simulink model "Guidance_HIL_XPlane"  (R2026b)
settings: Solver=ode4  StopTime=80  FixedStep=0.005  MaxStep=0.05  MinStep=1e-8  AbsTol=1e-4
StartFcn:
  | ins_initial_state_xplane;
undefined symbols (not defined in the file or in its folder): sensors
(part 2 of 2)

== matlab function Guidance_HIL_XPlane/Navigation/Error_Modeling/GPSNEO8M1/MATLAB Function ==
  data: pos_ned_true input; pos_em output; vel_ned_true input; t input; noise_pos_m input; noise_vel_ms input; w_bias_pos input; vel_em output
function [pos_em, vel_em] = gps_core(pos_ned_true, vel_ned_true, t, ...
    noise_pos_m, noise_vel_ms, w_bias_pos)
%#codegen

coder.extrinsic('ins_gps_measurements');
coder.extrinsic('evalin');

sensors = evalin('base', 'sensors');

y_gps = zeros(6,1);
tmp = zeros(6,1);

tmp = ins_gps_measurements(pos_ned_true, vel_ned_true, t, ...
    noise_pos_m, noise_vel_ms, w_bias_pos, sensors);

y_gps = tmp;

pos_em = y_gps(1:3);
vel_em = y_gps(4:6);

end

== matlab function Guidance_HIL_XPlane/Navigation/Error_Modeling/MAG-IST8310/MATLAB Function ==
  data: euler_true_rad input; yaw_mag_rad output; T input; noise_mag_uT input; mag_var input
function yaw_mag_rad = mag_core(euler_true_rad, T, noise_mag_uT, mag_var)
%#codegen

coder.extrinsic('ins_mag_meas');
coder.extrinsic('evalin');

sensors = evalin('base', 'sensors');

yaw_mag_rad = 0;
tmp = 0;

tmp = ins_mag_meas(euler_true_rad, T, noise_mag_uT, mag_var, sensors);

yaw_mag_rad = tmp;

end

== matlab function Guidance_HIL_XPlane/Navigation/Telemetry/MATLAB Function ==
  data: time input; h input; Vt input; V3D input; V3D_EKF input; cmds input; euler input
function ins_telemetry_block(time, h, Vt, V3D, V3D_EKF, cmds, euler)
%#codegen
% Wrapper para chamada extrinseca da telemetria no Simulink.

coder.extrinsic('ins_telemetry');

ins_telemetry(time, h, Vt, V3D, V3D_EKF, cmds, euler);

end

== matlab function Guidance_HIL_XPlane/Xplane Interface/X-Plane Sensors ==
  settings: updateMethod=DISCRETE  sampleTime=0.05
  data: xplane_sensors output; t input
function xplane_sensors = read_xplane_block(t)

coder.extrinsic('ins_read_xplane');

persistent y_last k_last

Ts_xplane = 0.05;

if isempty(y_last)
    y_last = zeros(1,18);
end

if isempty(k_last)
    k_last = -1;
end

% Índice discreto da interface X-Plane
k_now = floor(t / Ts_xplane + 1e-9);

% Por padrão, segura a última leitura
xplane_sensors = y_last;

% Só lê do X-Plane uma vez a cada Ts_xplane
if k_now > k_last
    tmp = zeros(1,18);
    tmp = ins_read_xplane(0);

    y_last = tmp;
    xplane_sensors = y_last;

    k_last = k_now;
end
end

== matlab function Guidance_HIL_XPlane/Navigation/MATLAB Function ==
  data: t_sil_xplane input; t_nav output; dt_xplane output; sample_valid output
function [t_nav, dt_xplane, sample_valid] = xplane_time_valid_block(t_sil_xplane)

persistent t0 t_prev initialized

if isempty(initialized)
    t0 = t_sil_xplane;
    t_prev = t_sil_xplane;
    initialized = true;
end

t_nav = t_sil_xplane - t0;
dt_xplane = t_sil_xplane - t_prev;

% Esperado: Ts_xplane ~= 0.05 s
% Aceita pequenas variações e rejeita amostras repetidas ou saltos absurdos
if dt_xplane > 1e-6 && dt_xplane < 0.20
    sample_valid = 1;
else
    sample_valid = 0;
end

if sample_valid == 1
    t_prev = t_sil_xplane;
end
end

== matlab function Guidance_HIL_XPlane/Navigation/Error_Modeling/ICM20689/gyro_core ==
  data: omega_meas_dps output double size=[3 1]; omega_true_dps input; T input; noise_dps input
function omega_meas_dps = gyro_core(omega_true_dps, T, noise_dps)
%#codegen

coder.extrinsic('ins_gyro_errors_icm20689');
coder.extrinsic('evalin');
sensors = evalin('base', 'sensors');
omega_meas_dps = zeros(3,1);
tmp = zeros(3,1);
tmp = ins_gyro_errors_icm20689(omega_true_dps, T, noise_dps, sensors);

omega_meas_dps = tmp;
end

== matlab function Guidance_HIL_XPlane/hil_io ==
  settings: updateMethod=DISCRETE  sampleTime=0.01
  data: sensors input double size=15; U1 output; U2 output; U3 output; U4 output
function [U1, U2, U3, U4] = hil_io(sensors)
%#codegen
U1 = 0; U2 = 0; U3 = 0; U4 = 0;
coder.extrinsic('hil_serial_step_guiagem');
s = sensors(:);
tmp = zeros(4,1);
tmp = hil_serial_step_guiagem(s);
U1 = tmp(1);
U2 = tmp(2);
U3 = tmp(3);
U4 = tmp(4);
end

== matlab function Guidance_HIL_XPlane/Xplane Interface/X-Plane Actuators ==
  settings: updateMethod=DISCRETE  sampleTime=0.05
  data: u input; t input; status output
function status = send_xplane_block(u, t)
%#codegen
coder.extrinsic('ins_send_xplane');
persistent k_last

Ts_xplane = 0.01;

if isempty(k_last)
    k_last = -1;
end

status = 0;

% Índice discreto da interface X-Plane
k_now = floor(t / Ts_xplane + 1e-9);

% Só envia comando uma vez a cada Ts_xplane
if k_now > k_last
    ins_send_xplane(u);

    k_last = k_now;
    status = 1;
end
end

== matlab function Guidance_HIL_XPlane/Navigation/Error_Modeling/ICM20689/acc_core ==
  data: acc_true_ms2 input double size=[3 1]; T input double size=[1 1]; noise_ms2 input; acc_meas_ms2 output double size=[3 1]
function acc_meas_ms2 = acc_core(acc_true_ms2, T, noise_ms2)
%#codegen

coder.extrinsic('ins_acc_errors_icm20689');
coder.extrinsic('evalin');

sensors = evalin('base', 'sensors');

acc_meas_ms2 = zeros(3,1);
tmp = zeros(3,1);

tmp = ins_acc_errors_icm20689(acc_true_ms2, T, noise_ms2, sensors);

acc_meas_ms2 = tmp;

end

== matlab function Guidance_HIL_XPlane/Navigation/DBN/MATLAB Function ==
  data: acc_b_in input; euler_out output; gyro_b_in input; reset input; sample_valid input; t_now input; vel_out output; pos_out output; acc_n_out output; qb_out output
function [euler_out, vel_out, pos_out, acc_n_out, qb_out] = DBN_block( ...
    acc_b_in, gyro_b_in, reset, sample_valid, t_now)
%#codegen

coder.extrinsic('DBN_solver');
coder.extrinsic('evalin');

euler_out = zeros(3,1);
vel_out   = zeros(3,1);
pos_out   = zeros(3,1);
acc_n_out = zeros(3,1);
qb_out    = zeros(4,1);

DBN_params = evalin('base', 'DBN_params');

euler_tmp = zeros(3,1);
vel_tmp   = zeros(3,1);
pos_tmp   = zeros(3,1);
acc_tmp   = zeros(3,1);
qb_tmp    = zeros(4,1);

[euler_tmp, vel_tmp, pos_tmp, acc_tmp, qb_tmp] = DBN_solver( ...
    acc_b_in, gyro_b_in, reset, sample_valid, t_now, DBN_params);

euler_out = euler_tmp;
vel_out   = vel_tmp;
pos_out   = pos_tmp;
acc_n_out = acc_tmp;
qb_out    = qb_tmp;

end

== matlab function Guidance_HIL_XPlane/Navigation/DBN/MATLAB Function1 ==
  data: acc_b_in input; euler_out output; gyro_b_in input; reset input; sample_valid input; t_now input; vel_out output; pos_out output; acc_n_out output; qb_out output
function [euler_out, vel_out, pos_out, acc_n_out, qb_out] = DBN_block_with_error_model( ...
    acc_b_in, gyro_b_in, reset, sample_valid, t_now)
%#codegen

coder.extrinsic('DBN_solver');
coder.extrinsic('evalin');

euler_out = zeros(3,1);
vel_out   = zeros(3,1);
pos_out   = zeros(3,1);
acc_n_out = zeros(3,1);
qb_out    = zeros(4,1);

DBN_params = evalin('base', 'DBN_params');

euler_tmp = zeros(3,1);
vel_tmp   = zeros(3,1);
pos_tmp   = zeros(3,1);
acc_tmp   = zeros(3,1);
qb_tmp    = zeros(4,1);

[euler_tmp, vel_tmp, pos_tmp, acc_tmp, qb_tmp] = DBN_solver( ...
    acc_b_in, gyro_b_in, reset, sample_valid, t_now, DBN_params);

euler_out = euler_tmp;
vel_out   = vel_tmp;
pos_out   = pos_tmp;
acc_n_out = acc_tmp;
qb_out    = qb_tmp;

end

== matlab function Guidance_HIL_XPlane/Navigation/EKFs/EKF_DIRETO ==
  data: acc_b_in input; euler_out output; vel_out output; pos_out output; gyro_b_in input; pos_meas_in input; vel_meas_in input; eul_meas_in input; reset input; sample_valid input; t_now input; acc_n_out output; xhat_out output
function [euler_out, vel_out, pos_out, acc_n_out, xhat_out] = EKF_DI_block( ...
    acc_b_in, gyro_b_in, pos_meas_in, vel_meas_in, eul_meas_in, reset, sample_valid, t_now)
%#codegen

coder.extrinsic('EKF_DI_solver');
coder.extrinsic('evalin');

%% Saídas com dimensão fixa

euler_out = zeros(3,1);
vel_out   = zeros(3,1);
pos_out   = zeros(3,1);
acc_n_out = zeros(3,1);
xhat_out  = zeros(21,1);

%% Variáveis temporárias com dimensão fixa

euler_tmp = zeros(3,1);
vel_tmp   = zeros(3,1);
pos_tmp   = zeros(3,1);
acc_tmp   = zeros(3,1);
xhat_tmp  = zeros(21,1);

%% Carrega parâmetros do workspace

EKF_DI_params = evalin('base', 'EKF_DI_params');

%% Chama solver externo

[euler_tmp, vel_tmp, pos_tmp, acc_tmp, xhat_tmp] = EKF_DI_solver( ...
    acc_b_in, gyro_b_in, pos_meas_in, vel_meas_in, eul_meas_in, ...
    reset, sample_valid, t_now, EKF_DI_params);

%% Cópia elemento a elemento para forçar dimensão no Simulink

euler_out(1) = euler_tmp(1);
euler_out(2) = euler_tmp(2);
euler_out(3) = euler_tmp(3);

vel_out(1) = vel_tmp(1);
vel_out(2) = vel_tmp(2);
vel_out(3) = vel_tmp(3);

pos_out(1) = pos_tmp(1);
pos_out(2) = pos_tmp(2);
pos_out(3) = pos_tmp(3);

acc_n_out(1) = acc_tmp(1);
acc_n_out(2) = acc_tmp(2);
acc_n_out(3) = acc_tmp(3);

for k = 1:21
    xhat_out(k) = xhat_tmp(k);
end

end
